simulink model "timedSpikingTemplate"  (R2026b)
settings: Solver=FixedStepAuto  StopTime=15  FixedStep=0.001
libraries: simulink x1, dspsigops x1
settings Model: Creator=40129232  LastModifiedBy=Eoin
settings DataIOCC: ReturnWorkspaceOutputs=off
settings OptimizationCC: LifeSpan=inf
settings DebuggingCC: ArithmeticOperatorsInVariantConditions=warning  SFExecutionAtInitializationDiag=none
settings SFSimCC: CustomCodeUndefinedFunction=UseInterfaceOnly  SimUseLocalCustomCode=off
settings RTWCC: DLArmComputeVersion=19.05  RTWUseLocalCustomCode=off
settings CodeAppCC: StateflowObjectComments=on

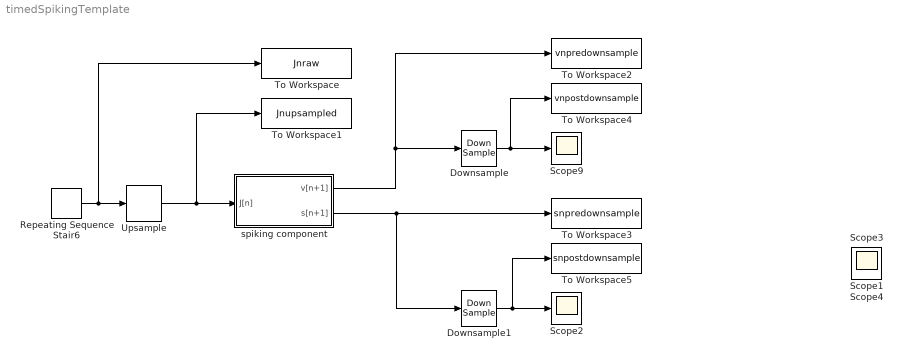
== system timedSpikingTemplate ==
  Downsample : DownSample  DownsamplingFactor=15
  Downsample1 : DownSample  DownsamplingFactor=15
  Repeating Sequence Stair6 : simulink/Sources/Repeating Sequence Stair  OutValues=[40.37, 52.35, 62.17, 70.19, 76.75].'  tsamp=0.015  OutMin=[]  OutMax=[]  OutDataTypeStr=double  OutputDataTypeScalingMode=double  OutDataType=fixdt(0,8)  ConRadixGroup=Best Precision: Vector-wise  OutScaling=2^-12
  Scope{1..4,9} (5 alike) : Scope
      Scope2 settings: ActiveDisplayYMinimum=-2.4434654473122719  ActiveDisplayYMaximum=3.9087776877612388
      Scope9 settings: ActiveDisplayYMinimum=-4.0597987314670611E+307  ActiveDisplayYMaximum=4.5108874794078445E+306  DataLoggingVariableName=ScopeData5
      Scope1 settings: ActiveDisplayYMinimum=-0.24987  ActiveDisplayYMaximum=2.24887
      Scope3 settings: ActiveDisplayYMinimum=-103.72127  ActiveDisplayYMaximum=38.33358  DataLoggingVariableName=ScopeData3
      Scope4 settings: ActiveDisplayYMinimum=-20.75486  ActiveDisplayYMaximum=56.79378  DataLoggingVariableName=ScopeData4
  To Workspace : ToWorkspace  VariableName=Jnraw  SaveFormat=Timeseries  SampleTime=-1
  To Workspace1 : ToWorkspace  VariableName=Jnupsampled  SaveFormat=Timeseries  SampleTime=-1
  To Workspace2 : ToWorkspace  VariableName=vnpredownsample  SaveFormat=Timeseries  SampleTime=-1
  To Workspace3 : ToWorkspace  VariableName=snpredownsample  SaveFormat=Timeseries  SampleTime=-1
  To Workspace4 : ToWorkspace  VariableName=vnpostdownsample  SaveFormat=Timeseries  SampleTime=-1
  To Workspace5 : ToWorkspace  VariableName=snpostdownsample  SaveFormat=Timeseries  SampleTime=-1
  Upsample : dspsigops/Upsample  FactorSource=Dialog parameter  UpsamplingFactor=15  MaxUpsamplingFactor=100  SampleOffset=0  RateOptions=Allow multirate processing  InitialConditions=0  mode=Unused parameter value
      settings: LibrarySourceBlock=dsphdlsupportsigops/Upsample
  spiking component : Subsystem
  wires:
  Downsample/1 -> To Workspace4/1, Scope9/1
  Downsample1/1 -> To Workspace5/1, Scope2/1
  Repeating Sequence Stair6/1 -> To Workspace/1, Upsample/1
  spiking component/2(s[n+1]) -> To Workspace3/1, Downsample1/1
  spiking component/1(v[n+1]) -> To Workspace2/1, Downsample/1
  Upsample/1 -> spiking component/1(J[n]), To Workspace1/1

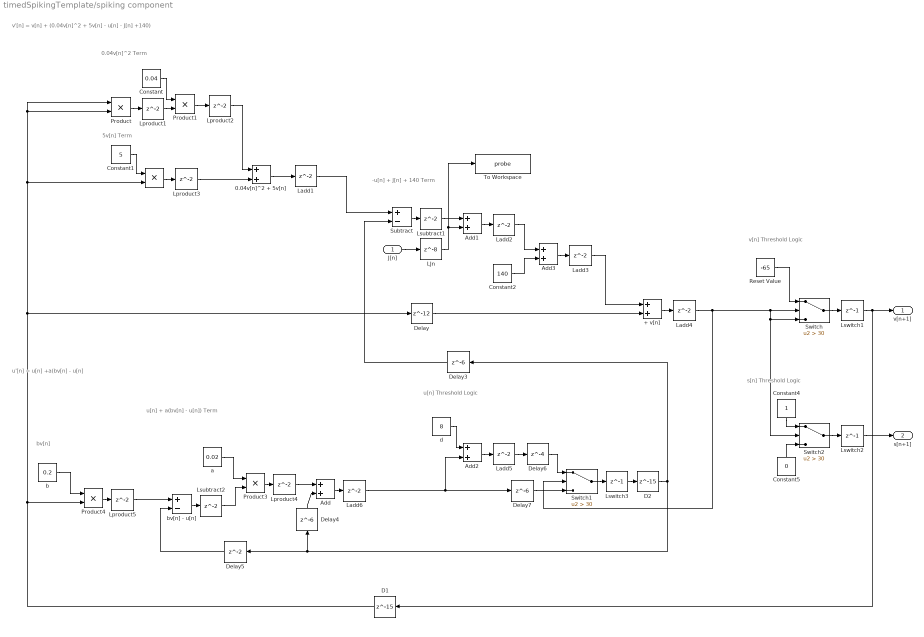
== system timedSpikingTemplate/spiking component ==
  note: u'[n] = u[n] +a(bv[n] - u[n]
  note: s[n] Threshold Logic
  note: u[n] Threshold Logic
  note: u[n] + a(bv[n] - u[n]) Term
  note: -u[n] + J[n] + 140 Term
  note: v[n] Threshold Logic
  note: bv[n]
  note: v'[n] = v[n] + (0.04v[n]^2 + 5v[n] - u[n] - J[n] +140)
  note: 5v[n] Term
  note: 0.04v[n]^2 Term
  J[n] : Inport  SampleTime=0.001
  " " : Product
  + v[n] : Sum
  0.04v[n]^2 + 5v[n] : Sum
  Add{,1..3} (4 alike) : Sum
  Constant : Constant  Value=0.04
  Constant1 : Constant  Value=5
  Constant2 : Constant  Value=140
  Constant4 : Constant
  Constant5 : Constant  Value=0
  D1 : Delay  DelayLength=15  InitialCondition=-65
  D2 : Delay  DelayLength=15  InitialCondition=0
  Delay : Delay  DelayLength=12  InitialCondition=0
  Delay3 : Delay  DelayLength=6  InitialCondition=0
  Delay4 : Delay  DelayLength=6  InitialCondition=0
  Delay5 : Delay  InitialCondition=0
  Delay6 : Delay  DelayLength=4  InitialCondition=0
  Delay7 : Delay  DelayLength=6  InitialCondition=0
  LJn : Delay  DelayLength=8  InitialCondition=0
  Ladd{1..6} (6 alike) : Delay  InitialCondition=0
  Lproduct{1..5} (5 alike) : Delay  InitialCondition=0
  Lsubtract1 : Delay  InitialCondition=0
  Lsubtract2 : Delay  InitialCondition=0
  Lswitch1 : Delay  DelayLength=1  InitialCondition=0
  Lswitch2 : Delay  DelayLength=1  InitialCondition=0
  Lswitch3 : Delay  DelayLength=1  InitialCondition=0
  Product{,1,3..4} (4 alike) : Product
  Reset Value : Constant  Value=-65
  Subtract : Sum  Inputs=+-
  Switch : Switch  Criteria=u2 > Threshold  Threshold=30  SaturateOnIntegerOverflow=off  InputSameDT=off
  Switch1 : Switch  Criteria=u2 > Threshold  Threshold=30  SaturateOnIntegerOverflow=off  InputSameDT=off
  Switch2 : Switch  Criteria=u2 > Threshold  Threshold=30  SaturateOnIntegerOverflow=off  InputSameDT=off
  To Workspace : ToWorkspace  VariableName=probe  SaveFormat=Timeseries  SampleTime=-1
  a : Constant  Value=0.02
  b : Constant  Value=0.2
  bv[n] - u[n] : Sum  Inputs=+-
  d : Constant  Value=8
  v[n+1] : Outport  VectorParamsAs1DForOutWhenUnconnected=off
  s[n+1] : Outport  Port=2  VectorParamsAs1DForOutWhenUnconnected=off
  wires:
  + v[n]/1 -> Ladd4/1
  Reset Value/1 -> Switch/1
  Constant1/1 -> " "/1
  Switch2/1 -> Lswitch2/1
  Constant5/1 -> Switch2/3
  Switch/1 -> Lswitch1/1
  Switch1/1 -> Lswitch3/1
  J[n]/1 -> LJn/1
  d/1 -> Add2/1
  Constant4/1 -> Switch2/1
  b/1 -> Product4/1
  Add/1 -> Ladd6/1
  Constant2/1 -> Add3/2
  a/1 -> Product3/1
  Constant/1 -> Product1/1
  Product/1 -> Lproduct1/1
  Lproduct1/1 -> Product1/2
  " "/1 -> Lproduct3/1
  0.04v[n]^2 + 5v[n]/1 -> Ladd1/1
  Ladd1/1 -> Subtract/1
  Subtract/1 -> Lsubtract1/1
  Lsubtract1/1 -> Add1/1
  Add1/1 -> Ladd2/1
  Ladd2/1 -> Add3/1
  Add3/1 -> Ladd3/1
  Ladd3/1 -> + v[n]/1
  Lswitch1/1 -> D1/1, v[n+1]/1
  Lswitch2/1 -> s[n+1]/1
  Product4/1 -> Lproduct5/1
  Lproduct5/1 -> bv[n] - u[n]/1
  Product3/1 -> Lproduct4/1
  Lproduct4/1 -> Add/1
  Lswitch3/1 -> D2/1
  Add2/1 -> Ladd5/1
  bv[n] - u[n]/1 -> Lsubtract2/1
  Lsubtract2/1 -> Product3/2
  Product1/1 -> Lproduct2/1
  Lproduct2/1 -> 0.04v[n]^2 + 5v[n]/1
  D1/1 -> Product4/2, Delay/1, Product/1, Product/2, " "/2
  Lproduct3/1 -> 0.04v[n]^2 + 5v[n]/2
  LJn/1 -> Add1/2, To Workspace/1
  Delay/1 -> + v[n]/2
  Delay3/1 -> Subtract/2
  D2/1 -> Delay5/1, Delay4/1, Delay3/1
  Delay4/1 -> Add/2
  Delay5/1 -> bv[n] - u[n]/2
  Ladd6/1 -> Delay7/1, Add2/2
  Delay7/1 -> Switch1/3
  Ladd4/1 -> Switch1/2, Switch/3, Switch2/2, Switch/2
  Ladd5/1 -> Delay6/1
  Delay6/1 -> Switch1/1
